simulink library "ConverterPlantLibrary"  (R2026a)
settings: Solver=VariableStepAuto
libraries: nesl_utility x213, fl_lib x211, ee_lib x205
(part 14 of 22)

== system ConverterPlantLibrary/Soft-Switching Converters/CLLC Converter/CLLCConverterVariant/SimplifiedModel/Resonant Tank/Vs ==
  PS-Simulink Converter : nesl_utility/PS-Simulink Converter  PhysicalDomain=network_engine_domain  SubClassName=ps_output  LeftPortType=input  RightPortType=output  PseudoPeriodic=off  Frequencies=[]  VectorFormat=inherit  Unit=inherit  AffineConversion=off
  Voltage Sensor : fl_lib/Electrical/Electrical Sensors/Voltage Sensor
  + : PMIOPort  Side=Left
  - : PMIOPort  Port=2  Side=Right
  V : Outport
  wires:
  PS-Simulink Converter/1 -> V/1
  connections:
  Voltage Sensor/RConn2 -- -/RConn1
  Voltage Sensor/LConn1 -- +/RConn1
  PS-Simulink Converter/LConn1 -- Voltage Sensor/RConn1

== system ConverterPlantLibrary/Soft-Switching Converters/CLLC Converter/CLLCConverterVariant/SimplifiedModel/Secondary Converter/Iout ==
  Current Sensor : fl_lib/Electrical/Electrical Sensors/Current Sensor
  PS-Simulink Converter : nesl_utility/PS-Simulink Converter  PhysicalDomain=network_engine_domain  SubClassName=ps_output  LeftPortType=input  RightPortType=output  PseudoPeriodic=off  Frequencies=[]  VectorFormat=inherit  Unit=inherit  AffineConversion=off
  + : PMIOPort  Side=Left
  - : PMIOPort  Port=2  Side=Right
  I : Outport
  wires:
  PS-Simulink Converter/1 -> I/1
  connections:
  Current Sensor/RConn2 -- -/RConn1
  +/RConn1 -- Current Sensor/LConn1
  Current Sensor/RConn1 -- PS-Simulink Converter/LConn1

== system ConverterPlantLibrary/Soft-Switching Converters/CLLC Converter/CLLCConverterVariant/SimplifiedModel/Secondary Converter/IoutRect ==
  Current Sensor : fl_lib/Electrical/Electrical Sensors/Current Sensor
  PS-Simulink Converter : nesl_utility/PS-Simulink Converter  PhysicalDomain=network_engine_domain  SubClassName=ps_output  LeftPortType=input  RightPortType=output  PseudoPeriodic=off  Frequencies=[]  VectorFormat=inherit  Unit=inherit  AffineConversion=off
  + : PMIOPort  Side=Left
  - : PMIOPort  Port=2  Side=Right
  I : Outport
  wires:
  PS-Simulink Converter/1 -> I/1
  connections:
  Current Sensor/RConn2 -- -/RConn1
  +/RConn1 -- Current Sensor/LConn1
  Current Sensor/RConn1 -- PS-Simulink Converter/LConn1

== system ConverterPlantLibrary/Soft-Switching Converters/CLLC Converter/CLLCConverterVariant/SimplifiedModel/Secondary Converter/Secondary Converter ==
  G1 : Inport
  G2 : Inport  Port=2
  G3 : Inport  Port=3
  G4 : Inport  Port=4
  MOSFETA1 : ee_lib/Semiconductors & Converters/Ideal Semiconductor Switch  port_option=ee.enum.controlport.ps  Ron=SecondaryRon Ohm  Goff=SecondaryGoff 1/Ohm  Vth=SecondaryVth V  diode_param=ee.enum.semiconductors.protectionDiode.nodynamics  diode_Vf=SecondaryVbodydiodeOn V  diode_Ron=SecondaryRbodydiodeOn Ohm  diode_Goff=SecondaryGbodydiodeOff 1/Ohm  diode_C=50e-9 F  diode_iRM=-235 A  diode_iF=300 A  diode_idot=-50 A/us  diode_trr_param=ee.enum.converters.diodetrr.trr_factor  diode_trr_factor=3  diode_trr=15 us  diode_Qrr=1500 s*uA
  MOSFETA2 : ee_lib/Semiconductors & Converters/Ideal Semiconductor Switch  port_option=ee.enum.controlport.ps  Ron=SecondaryRon Ohm  Goff=SecondaryGoff 1/Ohm  Vth=SecondaryVth V  diode_param=ee.enum.semiconductors.protectionDiode.nodynamics  diode_Vf=SecondaryVbodydiodeOn V  diode_Ron=SecondaryRbodydiodeOn Ohm  diode_Goff=SecondaryGbodydiodeOff 1/Ohm  diode_C=50e-9 F  diode_iRM=-235 A  diode_iF=300 A  diode_idot=-50 A/us  diode_trr_param=ee.enum.converters.diodetrr.trr_factor  diode_trr_factor=3  diode_trr=15 us  diode_Qrr=1500 s*uA
  MOSFETB1 : ee_lib/Semiconductors & Converters/Ideal Semiconductor Switch  port_option=ee.enum.controlport.ps  Ron=SecondaryRon Ohm  Goff=SecondaryGoff 1/Ohm  Vth=SecondaryVth V  diode_param=ee.enum.semiconductors.protectionDiode.nodynamics  diode_Vf=SecondaryVbodydiodeOn V  diode_Ron=SecondaryRbodydiodeOn Ohm  diode_Goff=SecondaryGbodydiodeOff 1/Ohm  diode_C=50e-9 F  diode_iRM=-235 A  diode_iF=300 A  diode_idot=-50 A/us  diode_trr_param=ee.enum.converters.diodetrr.trr_factor  diode_trr_factor=3  diode_trr=15 us  diode_Qrr=1500 s*uA
  MOSFETB2 : ee_lib/Semiconductors & Converters/Ideal Semiconductor Switch  port_option=ee.enum.controlport.ps  Ron=SecondaryRon Ohm  Goff=SecondaryGoff 1/Ohm  Vth=SecondaryVth V  diode_param=ee.enum.semiconductors.protectionDiode.nodynamics  diode_Vf=SecondaryVbodydiodeOn V  diode_Ron=SecondaryRbodydiodeOn Ohm  diode_Goff=SecondaryGbodydiodeOff 1/Ohm  diode_C=50e-9 F  diode_iRM=-235 A  diode_iF=300 A  diode_idot=-50 A/us  diode_trr_param=ee.enum.converters.diodetrr.trr_factor  diode_trr_factor=3  diode_trr=15 us  diode_Qrr=1500 s*uA
  Simulink-PS Converter{,1..3} (4 alike) : nesl_utility/Simulink-PS Converter  PhysicalDomain=network_engine_domain  SubClassName=ps_input  LeftPortType=input  RightPortType=output  PseudoPeriodic=off  Frequencies=[]  NoiseDistribution=none  NoiseParameters=[]  Unit=1  AffineConversion=off  FilteringAndDerivatives=provide  SimscapeFilterOrder=1  InputFilterTimeConstant=0.001  UdotUserProvided=0
  P1 : PMIOPort  Side=Right
  N1 : PMIOPort  Port=2  Side=Right
  P2 : PMIOPort  Port=3  Side=Left
  N2 : PMIOPort  Port=4  Side=Left
  wires:
  G1/1 -> Simulink-PS Converter/1
  G2/1 -> Simulink-PS Converter1/1
  G3/1 -> Simulink-PS Converter2/1
  G4/1 -> Simulink-PS Converter3/1
  connections:
  N2/RConn1 -- MOSFETB2/RConn1 -- MOSFETB1/RConn2
  P2/RConn1 -- MOSFETA2/RConn1 -- MOSFETA1/RConn2
  P1/RConn1 -- MOSFETB1/RConn1 -- MOSFETA1/RConn1
  N1/RConn1 -- MOSFETB2/RConn2 -- MOSFETA2/RConn2
  Simulink-PS Converter/RConn1 -- MOSFETA1/LConn1
  Simulink-PS Converter1/RConn1 -- MOSFETA2/LConn1
  Simulink-PS Converter2/RConn1 -- MOSFETB1/LConn1
  Simulink-PS Converter3/RConn1 -- MOSFETB2/LConn1

== system ConverterPlantLibrary/Soft-Switching Converters/CLLC Converter/CLLCConverterVariant/SimplifiedModel/Secondary Converter/Subsystem4 ==
  PS-Simulink Converter : nesl_utility/PS-Simulink Converter  PhysicalDomain=network_engine_domain  SubClassName=ps_output  LeftPortType=input  RightPortType=output  PseudoPeriodic=off  Frequencies=[]  VectorFormat=inherit  Unit=inherit  AffineConversion=off
  Voltage Sensor : fl_lib/Electrical/Electrical Sensors/Voltage Sensor
  + : PMIOPort  Side=Left
  - : PMIOPort  Port=2  Side=Right
  V : Outport
  wires:
  PS-Simulink Converter/1 -> V/1
  connections:
  Voltage Sensor/RConn2 -- -/RConn1
  Voltage Sensor/LConn1 -- +/RConn1
  PS-Simulink Converter/LConn1 -- Voltage Sensor/RConn1

== system ConverterPlantLibrary/Soft-Switching Converters/CLLC Converter/CLLCConverterVariant/SimplifiedModel/Secondary Converter/Vout ==
  PS-Simulink Converter : nesl_utility/PS-Simulink Converter  PhysicalDomain=network_engine_domain  SubClassName=ps_output  LeftPortType=input  RightPortType=output  PseudoPeriodic=off  Frequencies=[]  VectorFormat=inherit  Unit=inherit  AffineConversion=off
  Voltage Sensor : fl_lib/Electrical/Electrical Sensors/Voltage Sensor
  + : PMIOPort  Side=Left
  - : PMIOPort  Port=2  Side=Right
  V : Outport
  wires:
  PS-Simulink Converter/1 -> V/1
  connections:
  Voltage Sensor/RConn2 -- -/RConn1
  Voltage Sensor/LConn1 -- +/RConn1
  PS-Simulink Converter/LConn1 -- Voltage Sensor/RConn1

== system ConverterPlantLibrary/Soft-Switching Converters/DAB Converter/DABConverterVariant/DetailedModel/Lr/ExternalInductance ==
  Lr : fl_lib/Electrical/Electrical Elements/Inductor  l=Lr_SI H  r=RLr_SI Ohm  g=1e-05 1/Ohm  i_specify=off  i_priority=None  i=0 A  i_nominal_specify=off  i_nominal_value=1  i_nominal_unit=A  v_specify=off  v_priority=None  v=0 V  v_nominal_specify=off  v_nominal_value=1  v_nominal_unit=V  i_L_specify=off  i_L_priority=High  i_L=0 A  i_L_nominal_specify=off  i_L_nominal_value=1  i_L_nominal_unit=A
  P : PMIOPort  Side=Left
  N : PMIOPort  Port=2  Side=Right
  connections:
  P/RConn1 -- Lr/LConn1
  Lr/RConn1 -- N/RConn1

== system ConverterPlantLibrary/Soft-Switching Converters/DAB Converter/DABConverterVariant/DetailedModel/Lr/LeakageInductance ==
  P : PMIOPort  Side=Left
  N : PMIOPort  Port=2  Side=Right
  connections:
  P/RConn1 -- N/RConn1

== system ConverterPlantLibrary/Soft-Switching Converters/DAB Converter/DABConverterVariant/DetailedModel/PrimaryBridge/IdealSwitch ==
  G : Inport
  Demux : Demux
  MOSFETPriA1 : ee_lib/Semiconductors & Converters/Ideal Semiconductor Switch  port_option=ee.enum.controlport.ps  Ron=RdsOnPri_SI Ohm  Goff=GdsOffPri_SI 1/Ohm  Vth=VthPri_SI V  diode_param=ee.enum.semiconductors.protectionDiode.nodynamics  diode_Vf=VfPri_SI V  diode_Ron=RdPri_SI Ohm  diode_Goff=GdPri_SI 1/Ohm  diode_C=50e-9 F  diode_iRM=-235 A  diode_iF=300 A  diode_idot=-50 A/us  diode_trr_param=ee.enum.converters.diodetrr.trr_factor  diode_trr_factor=3  diode_trr=15 us  diode_Qrr=1500 s*uA
  MOSFETPriA2 : ee_lib/Semiconductors & Converters/Ideal Semiconductor Switch  port_option=ee.enum.controlport.ps  Ron=RdsOnPri_SI Ohm  Goff=GdsOffPri_SI 1/Ohm  Vth=VthPri_SI V  diode_param=ee.enum.semiconductors.protectionDiode.nodynamics  diode_Vf=VfPri_SI V  diode_Ron=RdPri_SI Ohm  diode_Goff=GdPri_SI 1/Ohm  diode_C=50e-9 F  diode_iRM=-235 A  diode_iF=300 A  diode_idot=-50 A/us  diode_trr_param=ee.enum.converters.diodetrr.trr_factor  diode_trr_factor=3  diode_trr=15 us  diode_Qrr=1500 s*uA
  MOSFETPriB1 : ee_lib/Semiconductors & Converters/Ideal Semiconductor Switch  port_option=ee.enum.controlport.ps  Ron=RdsOnPri_SI Ohm  Goff=GdsOffPri_SI 1/Ohm  Vth=VthPri_SI V  diode_param=ee.enum.semiconductors.protectionDiode.nodynamics  diode_Vf=VfPri_SI V  diode_Ron=RdPri_SI Ohm  diode_Goff=GdPri_SI 1/Ohm  diode_C=50e-9 F  diode_iRM=-235 A  diode_iF=300 A  diode_idot=-50 A/us  diode_trr_param=ee.enum.converters.diodetrr.trr_factor  diode_trr_factor=3  diode_trr=15 us  diode_Qrr=1500 s*uA
  MOSFETPriB2 : ee_lib/Semiconductors & Converters/Ideal Semiconductor Switch  port_option=ee.enum.controlport.ps  Ron=RdsOnPri_SI Ohm  Goff=GdsOffPri_SI 1/Ohm  Vth=VthPri_SI V  diode_param=ee.enum.semiconductors.protectionDiode.nodynamics  diode_Vf=VfPri_SI V  diode_Ron=RdPri_SI Ohm  diode_Goff=GdPri_SI 1/Ohm  diode_C=50e-9 F  diode_iRM=-235 A  diode_iF=300 A  diode_idot=-50 A/us  diode_trr_param=ee.enum.converters.diodetrr.trr_factor  diode_trr_factor=3  diode_trr=15 us  diode_Qrr=1500 s*uA
  SL_PS{1..4} (4 alike) : nesl_utility/Simulink-PS Converter  PhysicalDomain=network_engine_domain  SubClassName=ps_input  LeftPortType=input  RightPortType=output  PseudoPeriodic=off  Frequencies=[]  NoiseDistribution=none  NoiseParameters=[]  Unit=1  AffineConversion=off  FilteringAndDerivatives=provide  SimscapeFilterOrder=1  InputFilterTimeConstant=0.001  UdotUserProvided=0
  VinP : PMIOPort  Side=Left
  VinN : PMIOPort  Port=2  Side=Left
  MidA : PMIOPort  Port=3  Side=Right
  MidB : PMIOPort  Port=4  Side=Right
  wires:
  [G4] -> SL_PS4/1
  [G3] -> SL_PS3/1
  [G2] -> SL_PS2/1
  [G1] -> SL_PS1/1
  Demux/4 -> [G4]
  Demux/3 -> [G3]
  Demux/2 -> [G2]
  Demux/1 -> [G1]
  G/1 -> Demux/1
  connections:
  MOSFETPriA2/RConn2 -- MOSFETPriB2/RConn2 -- VinN/RConn1
  MidA/RConn1 -- MOSFETPriA2/RConn1 -- MOSFETPriA1/RConn2
  MOSFETPriB2/RConn1 -- MidB/RConn1 -- MOSFETPriB1/RConn2
  MOSFETPriB1/RConn1 -- MOSFETPriA1/RConn1 -- VinP/RConn1
  SL_PS1/RConn1 -- MOSFETPriA1/LConn1
  SL_PS2/RConn1 -- MOSFETPriA2/LConn1
  SL_PS3/RConn1 -- MOSFETPriB1/LConn1
  SL_PS4/RConn1 -- MOSFETPriB2/LConn1
